simulink model "FAFA_Simulation"  (R2024b)
settings: Solver=FixedStepAuto  StartTime=0.0  StopTime=250  FixedStep=0.1  RelTol=1e-3
model workspace (MAT data in the model file):
  E = 0
  N = 0
  U = 70
  a_lat = [-2.8994  0.2017  -1.4522  -1.3994; -3.7694  1.1605  0.9879  -0.5752; 4.8979  -2.4536  -4.2099  -0.5761; 0.9075  1.8506  6.4665  2.8087]
  a_lon = [-0.1636  -0.7164  0.3908  0.5329; 0.8185  -0.2899  2.1971  2.5997; -0.1448  -2.0395  -0.2446  1.4062; 0.6823  -2.5415  -6.117  -5.7482]
  b_lat = [-2.6641  1.8404; -6.8743  1.3852; 17.3529  -0.0089; -11.8089  -3.3692]
  b_lon = [1.3105; 2.2437; -0.9608; -9.211]
  c_lat = [-0.6923  0.0805  -0.3221  -0.3931; -1.1619  0.5751  1.1098  0.0833; 0.5476  0.4203  0.2079  -0.0052; -0.4273  0.7792  0.2479  -0.0005]
  c_lon = [-5.1576  -28.9963  19.7487  -10.7497; -0.0952  -0.3715  -0.0997  -0.0942; 0.5331  -3.4973  -0.5832  0.4945; 3.6707  -0.1414  -0.2256  -0.1149]
  d_lat = [0  0; 0  0; 0  0; 0  0]
  d_lon = [0; 0; 0; 0]
  psi0 = 0
  wind_E0 = 0
  wind_N0 = 0
  wind_heading = 100
  wind_noise = 0
  wind_turbulance_value0 = 1
  wind_value0 = 0
  x0_lat = [0; 0; 0; 0]
  x0_lon = [0; 0; 0; 0]
undefined symbols (not defined in the file): dspblkCoreblockFVToolHelper, F, gcbh, Light, MIL, velocity, waypoints
libraries: simulink x8, slpidlib x5, aerolibwind2 x3, sharedtransform x2, rllib x1, uavutilslib x1
(part 1 of 3)
settings Model: PacingRate=3  Creator=user  LastModifiedBy=yeyi5
settings DataIOCC: SaveOutput=off  SignalLogging=off  DSMLogging=off  SaveTime=off
settings OptimizationCC: ReuseModelBlockBuffer=off
settings DebuggingCC: AlgebraicLoopMsg=none  ArtificialAlgebraicLoopMsg=none  InheritedTsInSrcMsg=none  TasksWithSamePriorityMsg=none  SigSpecEnsureSampleTimeMsg=none  UnconnectedLineMsg=warning  UnknownTsInhSupMsg=none  ModelReferenceDataLoggingMessage=none  OperatingPointInterfaceChecksumMismatchMsg=none  SFUnusedDataAndEventsDiag=none  SFTransitionActionBeforeConditionDiag=none  IntegerSaturationMsg=none
settings ModelReferenceCC: EnableRefExpFcnMdlSchedulingChecks=on
settings RTWCC: GPUComputeCapability=3.5  DLArmComputeVersion=19.05

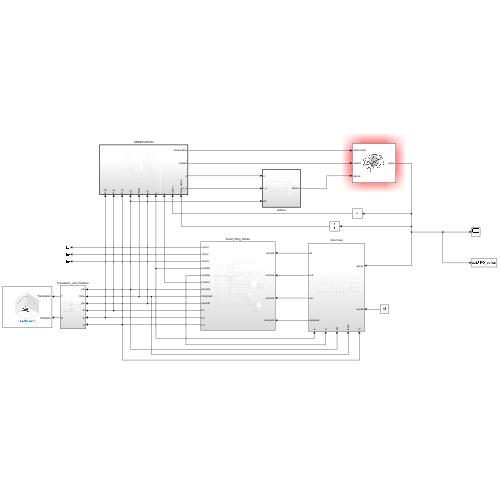
[thumbnail: Simulink's stored preview of the top-level diagram]
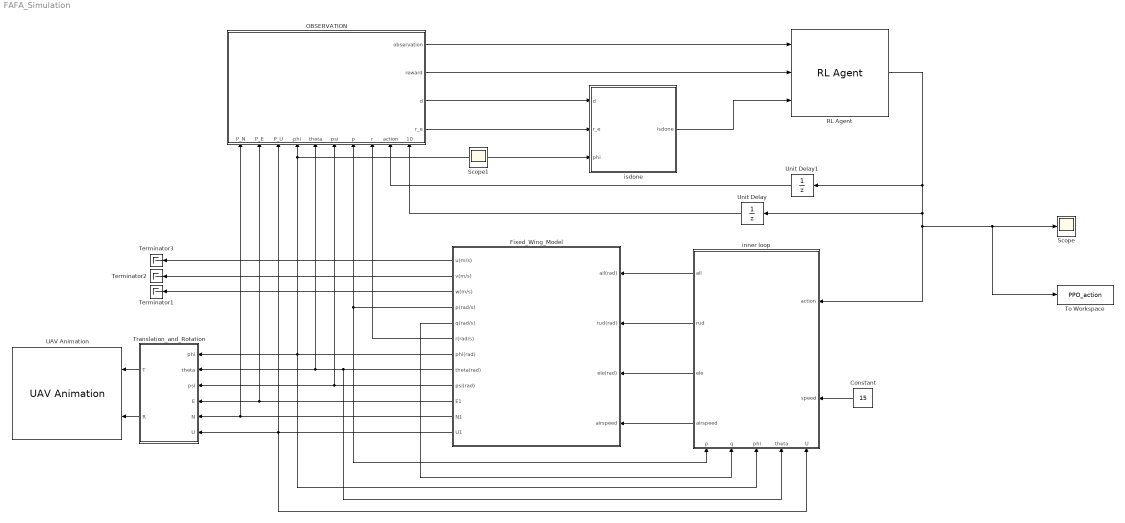
== system FAFA_Simulation ==
  Constant : Constant  Value=15
  Fixed_Wing_Model : Subsystem
  OBSERVATION : Subsystem  TreatAsAtomicUnit=on
      settings: PortSchema="{\"entries\":[{\"content\":{\"sides\":[{\"content\":{},\"type\":\"ConnectorPlacement.EquallySpacedRectSide\",\"uuid\":\"f286f6f9-a01a-42a6-836e-b598d67e253d\"},{\"content\":{\"connectorIds\":[\"Out1\",\"Out2\",\"Out3\",\"Out4\"],\"side\":\"RIGHT\"},\"type\":\"ConnectorPlacement.EquallySpacedRectSide\",\"uuid\":\"2d728f1a-8a2e-4ecd-bbb7-96377896084d\"},{\"content\":{\"side\":\"TOP\"},\"type\":\"ConnectorPlacement.EquallySpacedRectSide\",\"uuid\":\"cacb8353-56c3-4403-9fcf-3680ca0986aa\"},{\"content\":{\"connectorIds\":[\"In1\",\"In2\",\"In3\",\"In4\",\"In5\",\"In6\",\"In7\",\"In8\",\"In9\",\"In10\"],\"side\":\"BOTTOM\"},\"type\":\"ConnectorPlacement.EquallySpacedRectSide\",\"uuid\":\"73d02477-6798-4d99-8273-17e2202a1dc5\"}]},\"type\":\"ConnectorPlacement.EquallySpacedConnector\",\"uuid\":\"e5ed1a66-3715-4ac1-9ed0-cc3d392d34e5\"}],\"packageUris\":[\"http://schema.mathworks.com/mf0/Connector/R2020b\"],\"version\":\"1.0\"}"
  RL Agent : rllib/RL Agent  Agent=Agent_Stage2  ExternalActionAsInput=off  ProvideLastAction=off  ProvideCumRwd=off  TreatAsDirectFeedthrough=on  UseStrictObservationDataTypes=off
  Scope : Scope
  Terminator1 : Terminator
  Terminator2 : Terminator
  Terminator3 : Terminator
  To Workspace : ToWorkspace  VariableName=PPO_action  SaveFormat=Timeseries  SampleTime=-1
  Translation_and_Rotation : Subsystem
  UAV Animation : uavutilslib/UAV Animation  NumUAV=1  DynamicUAVConfig=off  UAVType=FixedWing  UAVSize=50  UAVColor=[1 0 0]  UAVTrajectoryAlpha=1  InertialZDirection=Up  RotationFormat=Quaternion  DrawMarkers=off  SampleTime=0.1
  Unit Delay : UnitDelay  SampleTime=0.2  HasFrameUpgradeWarning=on
  Unit Delay1 : UnitDelay  SampleTime=0.1  HasFrameUpgradeWarning=on
  inner loop : Subsystem
      settings: PortSchema="{\"entries\":[{\"content\":{\"sides\":[{\"content\":{\"connectorIds\":[\"In1\",\"In2\"]},\"type\":\"ConnectorPlacement.EquallySpacedRectSide\",\"uuid\":\"7d60b91c-7846-4215-9a9d-48d8590b6647\"},{\"content\":{\"connectorIds\":[\"Out1\",\"Out2\",\"Out3\",\"Out4\"],\"side\":\"RIGHT\"},\"type\":\"ConnectorPlacement.EquallySpacedRectSide\",\"uuid\":\"9adb366d-c473-491f-8767-4ec8db5c324b\"},{\"content\":{\"connectorIds\":[\"In3\",\"In4\",\"In5\",\"In6\",\"In7\"],\"side\":\"TOP\"},\"type\":\"ConnectorPlacement.EquallySpacedRectSide\",\"uuid\":\"05cfcaa8-de81-40d5-bf1e-81a0cec58454\"},{\"content\":{\"side\":\"BOTTOM\"},\"type\":\"ConnectorPlacement.EquallySpacedRectSide\",\"uuid\":\"953cf2cb-5cfd-4159-a7f8-9598cb97629a\"}]},\"type\":\"ConnectorPlacement.EquallySpacedConnector\",\"uuid\":\"4935b2dc-fa79-4ba1-b3ea-575a125b9ddc\"}],\"packageUris\":[\"http://schema.mathworks.com/mf0/Connector/R2020b\"],\"version\":\"1.0\"}"
  isdone : Subsystem  TreatAsAtomicUnit=on
  Scope1 : Scope
  wires:
  Translation_and_Rotation/2(R) -> UAV Animation/2
  Translation_and_Rotation/1(T) -> UAV Animation/1
  Fixed_Wing_Model/3(w(m/s)) -> Terminator1/1
  Fixed_Wing_Model/2(v(m/s)) -> Terminator2/1
  Fixed_Wing_Model/1(u(m/s)) -> Terminator3/1
  RL Agent/1 -> Unit Delay1/1, Scope/1, To Workspace/1, inner loop/2(action), Unit Delay/1
  OBSERVATION/2(reward) -> RL Agent/2
  OBSERVATION/1(observation) -> RL Agent/1
  OBSERVATION/3(d) -> isdone/1(d)
  OBSERVATION/4(r_e) -> isdone/2(r_e)
  Fixed_Wing_Model/4(p(rad/s)) -> inner loop/7(p), OBSERVATION/7(p)
  Fixed_Wing_Model/5(q(rad/s)) -> inner loop/6(q)
  Fixed_Wing_Model/6(r(rad/s)) -> OBSERVATION/8(r)
  Fixed_Wing_Model/7(phi(rad)) -> inner loop/5(phi), Translation_and_Rotation/1(phi), isdone/3(phi), OBSERVATION/4(phi)
  Fixed_Wing_Model/8(theta(rad)) -> OBSERVATION/5(theta), Translation_and_Rotation/2(theta), inner loop/4(theta)
  Fixed_Wing_Model/9(psi(rad)) -> Translation_and_Rotation/3(psi), OBSERVATION/6(psi)
  Fixed_Wing_Model/10(E1) -> Translation_and_Rotation/4(E), OBSERVATION/2(P_E)
  Fixed_Wing_Model/11(N1) -> Translation_and_Rotation/5(N), OBSERVATION/1(P_N)
  Fixed_Wing_Model/12(U1) -> inner loop/3(U), Translation_and_Rotation/6(U), OBSERVATION/3(P_U)
  Unit Delay1/1 -> OBSERVATION/9(action)
  Unit Delay/1 -> OBSERVATION/10(delay_action)
  inner loop/4(ail) -> Fixed_Wing_Model/1(ail(rad))
  inner loop/3(rud) -> Fixed_Wing_Model/2(rud(rad))
  inner loop/2(ele) -> Fixed_Wing_Model/3(ele(rad))
  inner loop/1(airspeed) -> Fixed_Wing_Model/4(airspeed)
  Constant/1 -> inner loop/1(speed)
  isdone/1(isdone) -> RL Agent/3

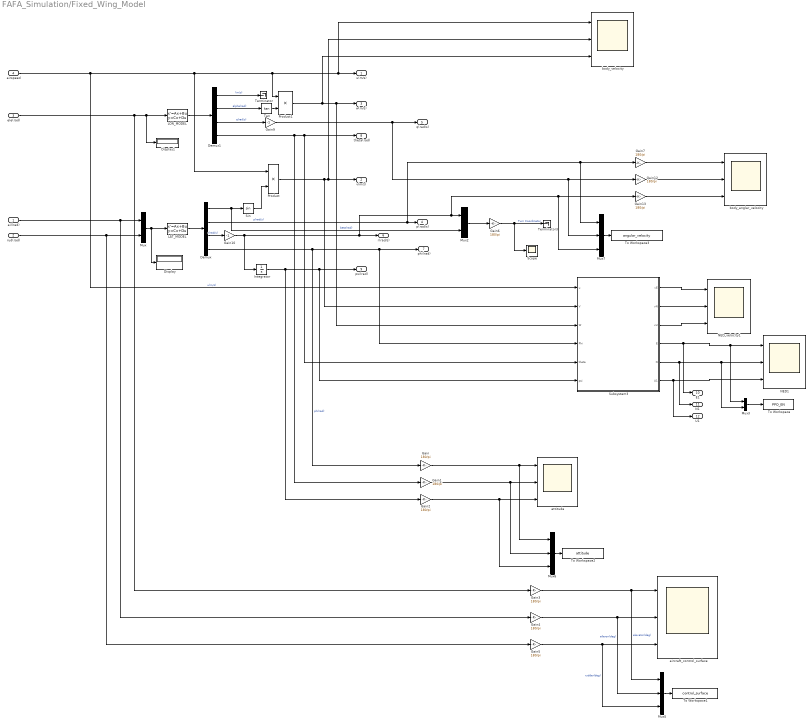
== system FAFA_Simulation/Fixed_Wing_Model ==
  ail(rad) : Inport
  rud(rad) : Inport  Port=2
  ele(rad) : Inport  Port=3
  airspeed : Inport  Port=4
  Demux : Demux
  Demux1 : Demux
  Display : Display
  Display1 : Display
  Gain{,1..7,12..13} (10 alike) : Gain  Gain=180/pi
  Gain10 : Gain  Gain=-1
  Gain9 : Gain  Gain=-1
  Integrator : Integrator  InitialCondition=psi0  WrapState=on
  LAT_MODEL : StateSpace  A=a_lat  B=b_lat  C=c_lat  D=d_lat  InitialCondition=x0_lat
  LON_MODEL : StateSpace  A=a_lon  B=b_lon  C=c_lon  D=d_lon  InitialCondition=x0_lon
  Mux : Mux  Inputs=2
  Mux2 : Mux  Inputs=2
  Mux3 : Mux  Inputs=2
  Mux5 : Mux  Inputs=3
  Mux6 : Mux  Inputs=3
  Mux7 : Mux  Inputs=3
  NED1 : Scope  NumInputPorts=3
  NED_velocity1 : Scope  NumInputPorts=3
  Product : Product
  Product1 : Product
  Scope : Scope
  Sin : Trigonometry
  Subsystem3 : Subsystem
  Tan : Trigonometry  Operator=tan
  Terminator : Terminator
  Terminator3 : Terminator
  To Workspace : ToWorkspace  VariableName=PPO_EN  SaveFormat=Timeseries  SampleTime=-1
  To Workspace1 : ToWorkspace  VariableName=control_surface  SaveFormat=Timeseries  SampleTime=-1
  To Workspace2 : ToWorkspace  VariableName=attitude  SaveFormat=Timeseries  SampleTime=-1
  To Workspace3 : ToWorkspace  VariableName=angular_velocity  SaveFormat=Timeseries  SampleTime=-1
  aircraft_control_surface : Scope  NumInputPorts=3
  attitude : Scope  NumInputPorts=3
  body_anglar_velocity : Scope  NumInputPorts=3
  body_velocity : Scope  NumInputPorts=3
  u(m/s) : Outport
  v(m/s) : Outport  Port=2
  w(m/s) : Outport  Port=3
  p(rad/s) : Outport  Port=4
  q(rad/s) : Outport  Port=5
  r(rad/s) : Outport  Port=6
  phi(rad) : Outport  Port=7
  theta(rad) : Outport  Port=8
  psi(rad) : Outport  Port=9
  E1 : Outport  Port=10
  N1 : Outport  Port=11
  U1 : Outport  Port=12
  wires:
  Demux/3 -> Gain10/1  "r(rad/s)"
  Mux/1 -> Display/1, LAT_MODEL/1
  LON_MODEL/1 -> Demux1/1
  Demux/1 -> Sin/1, Mux2/2  "beta(rad)"
  LAT_MODEL/1 -> Demux/1
  Demux/2 -> Mux7/1, Gain7/1, p(rad/s)/1  "p(rad/s)"
  airspeed/1 -> Subsystem3/1(u), body_velocity/1, u(m/s)/1, Product1/1, Product/1  "u(m/s)"
  Sin/1 -> Product/2
  Demux1/1 -> Terminator/1  "(m/s)"
  Demux1/2 -> Tan/1  "alpha(rad)"
  Demux1/3 -> Gain9/1  "q(rad/s)"
  Tan/1 -> Product1/2
  Gain/1 -> Mux6/1, attitude/1
  Gain1/1 -> Mux6/2, attitude/2
  Gain5/1 -> Mux5/3, aircraft_control_surface/3  "rudder(deg)"
  Gain3/1 -> Mux5/1, aircraft_control_surface/1  "elevator(deg)"
  Gain4/1 -> Mux5/2, aircraft_control_surface/2  "aileron(deg)"
  Mux5/1 -> To Workspace1/1
  Mux6/1 -> To Workspace2/1
  Mux7/1 -> To Workspace3/1
  Mux2/1 -> Gain6/1
  Gain6/1 -> Scope/1, Terminator3/1  "Turn Coordinator"
  Demux/4 -> Subsystem3/4(Phi), phi(rad)/1, Gain/1  "phi(rad)"
  Subsystem3/1(vE) -> NED_velocity1/1
  Subsystem3/2(vN) -> NED_velocity1/2
  Subsystem3/3(vU) -> NED_velocity1/3
  Gain9/1 -> Mux7/2, Gain12/1, q(rad/s)/1
  Gain2/1 -> Mux6/3, attitude/3
  Mux3/1 -> To Workspace/1
  Integrator/1 -> Subsystem3/6(psi), psi(rad)/1, Gain2/1
  Gain10/1 -> r(rad/s)/1, Mux7/3, Gain13/1, Mux2/1, Integrator/1
  Gain7/1 -> body_anglar_velocity/1
  Gain12/1 -> body_anglar_velocity/2
  Gain13/1 -> body_anglar_velocity/3
  ail(rad)/1 -> Gain4/1, Mux/1
  rud(rad)/1 -> Gain5/1, Mux/2
  Subsystem3/4(E) -> E1/1, Mux3/1, NED1/1
  Subsystem3/5(N) -> N1/1, Mux3/2, NED1/2
  Subsystem3/6(U1) -> U1/1, NED1/3
  Product/1 -> Subsystem3/2(V), v(m/s)/1, body_velocity/2
  Product1/1 -> body_velocity/3, Subsystem3/3(W), w(m/s)/1
  Demux1/4 -> theta(rad)/1, Subsystem3/5(theta), Gain1/1
  ele(rad)/1 -> Gain3/1, Display1/1, LON_MODEL/1

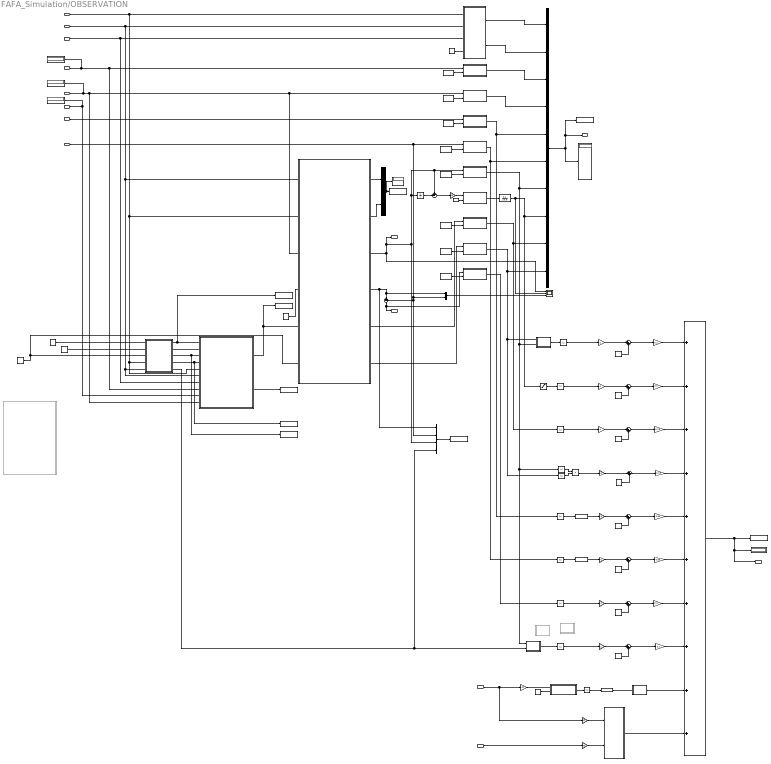
== system FAFA_Simulation/OBSERVATION ==
  P_N : Inport
  P_E : Inport  Port=2
  P_U : Inport  Port=3
  phi : Inport  Port=4
  theta : Inport  Port=5
  psi : Inport  Port=6
  p : Inport  Port=7
  r : Inport  Port=8
  action : Inport  Port=9
  delay_action : Inport  Port=10
  Abs{1,3..5,10..13,15,17} (10 alike) : Abs  SaturateOnIntegerOverflow=off
  Compare To Constant2 : simulink/Logic and Bit Operations/Compare To Constant  relop=>=  const=0.5  OutDataTypeStr=boolean
  Compare To Constant5 : simulink/Logic and Bit Operations/Compare To Constant  relop=>=  const=0.5  OutDataTypeStr=boolean
  Compare To Constant7 : simulink/Logic and Bit Operations/Compare To Constant  relop=>  const=1  OutDataTypeStr=boolean
  Constant : Constant  Value=15
  Constant1 : Constant  Value=60*pi/180
  Constant10 : Constant  Value=30
  Constant11 : Constant  Value=6
  Constant12 : Constant  Value=pi
  Constant{13,16,18..22,24} (8 alike) : Constant
  Constant14 : Constant  Value=1/55
  Constant15 : Constant  Value=25*pi/180
  Constant2 : Constant  Value=60*pi/180
  Constant27 : Constant  Value=40
  Constant4 : Constant  Value=100
  Constant7 : Constant  Value=0.01
  Constant8 : Constant  Value=40*pi/180
  Constant9 : Constant  Value=pi/2
  Discrete Transfer Fcn : DiscreteTransferFcn  LoadFcn=dspblkCoreblockFVToolHelper(gcbh,'load');  Numerator=[0.2]  Denominator=[1, -0.8]
      settings: CopyFcn=dspblkCoreblockFVToolHelper(gcbh,'copy');  DeleteFcn=dspblkCoreblockFVToolHelper(gcbh,'close');  ModelCloseFcn=dspblkCoreblockFVToolHelper(gcbh,'close');  PreSaveFcn=dspblkCoreblockFVToolHelper(gcbh,'presave');  PostSaveFcn=dspblkCoreblockFVToolHelper(gcbh,'postsave');  CloseFcn=dspblkCoreblockFVToolHelper(gcbh,'close');
  Display{,1..5} (6 alike) : Display
  Gain{1,10,14..16,21..22} (7 alike) : Gain  Gain=-1
  Gain11 : Gain  Gain=0.1
  Gain12 : Gain
  Gain13 : Gain  Gain=0.1
  Gain17 : Gain  Gain=0.15
  Gain18 : Gain  Gain=0.05
  Gain19 : Gain  Gain=0.2
  Gain20 : Gain  Gain=0.15
  Gain23 : Gain  Gain=0.05
  Gain4 : Gain  Gain=40
  Gain5 : Gain  Gain=40
  Gain6 : Gain  Gain=40
  Gain8 : Gain  Gain=10
  Gain9 : Gain  Gain=0.2
  MATLAB Function1 : MATLAB Function  TreatAsAtomicUnit=on
  MATLAB Function10 : MATLAB Function  TreatAsAtomicUnit=on
  MATLAB Function11 : MATLAB Function  TreatAsAtomicUnit=on
  MATLAB Function12 : MATLAB Function  TreatAsAtomicUnit=on  SystemSampleTime=0.1
  MATLAB Function13 : MATLAB Function  TreatAsAtomicUnit=on
  MATLAB Function14 : MATLAB Function  Commented=on  TreatAsAtomicUnit=on
  MATLAB Function15 : MATLAB Function  TreatAsAtomicUnit=on
  MATLAB Function16 : MATLAB Function  TreatAsAtomicUnit=on
  MATLAB Function18 : MATLAB Function  TreatAsAtomicUnit=on
  MATLAB Function2 : MATLAB Function  TreatAsAtomicUnit=on
  MATLAB Function20 : MATLAB Function  TreatAsAtomicUnit=on
  MATLAB Function21 : MATLAB Function  Commented=on  TreatAsAtomicUnit=on
  MATLAB Function22 : MATLAB Function  TreatAsAtomicUnit=on
  MATLAB Function3 : MATLAB Function  TreatAsAtomicUnit=on  SystemSampleTime=0.1
  MATLAB Function4 : MATLAB Function  TreatAsAtomicUnit=on
  MATLAB Function5 : MATLAB Function  TreatAsAtomicUnit=on
  MATLAB Function6 : MATLAB Function  TreatAsAtomicUnit=on
  MATLAB Function7 : MATLAB Function  TreatAsAtomicUnit=on
  MATLAB Function8 : MATLAB Function  TreatAsAtomicUnit=on  SystemSampleTime=0.1
  MATLAB Function9 : MATLAB Function  TreatAsAtomicUnit=on
  Mux : Mux  Inputs=10
  Mux1 : Mux  Inputs=2
  Mux2 : Mux
  Mux3 : Mux  Inputs=2
  Product : Product
  Saturation : Saturate  UpperLimit=1  LowerLimit=-1
  Straight Line V4 : MATLAB Function  Commented=on  TreatAsAtomicUnit=on  SystemSampleTime=0.1
  Sum : Sum  Inputs=|+-
  Sum{4..5,7,10..14} (8 alike) : Sum  Inputs=|++
  Sum3 : Sum  Inputs=++++++++++
  Sum6 : Sum  Inputs=+-|
  To Workspace1 : ToWorkspace  VariableName=PPO_ref_EN  SaveFormat=Timeseries  SampleTime=-1
  To Workspace2 : ToWorkspace  VariableName=SPSO_path  SaveFormat=Timeseries  SampleTime=-1
  To Workspace3 : ToWorkspace  VariableName=Reward  SaveFormat=Timeseries  SampleTime=-1
  To Workspace4 : ToWorkspace  VariableName=observation  SaveFormat=Timeseries  SampleTime=-1
  To Workspace5 : ToWorkspace  VariableName=valid_flag  SaveFormat=Timeseries  SampleTime=-1
  To Workspace6 : ToWorkspace  VariableName=loiter_flag  SaveFormat=Timeseries  SampleTime=-1
  To Workspace7 : ToWorkspace  VariableName=target_trajectory  SaveFormat=Timeseries  SampleTime=-1
  To Workspace8 : ToWorkspace  VariableName=guidance_error  SaveFormat=Timeseries  SampleTime=-1
  To Workspace9 : ToWorkspace  VariableName=guidance_mode  SaveFormat=Timeseries  SampleTime=-1
  Unit Delay : UnitDelay  SampleTime=0.1  HasFrameUpgradeWarning=on
  guidance_error : Scope  NumInputPorts=3
  velocity : Constant  Value=velocity
  waypoints : Constant  Value=waypoints
  observation : Outport
  reward : Outport  Port=2
  d : Outport  Port=3
  r_e : Outport  Port=4
  wires:
  Gain15/1 -> Sum10/1
  Sum10/1 -> Gain9/1
  Abs10/1 -> Gain15/1  "d"
  Constant18/1 -> Sum10/2
  Gain16/1 -> Sum11/1
  Sum11/1 -> Gain17/1
  Constant20/1 -> Sum11/2
  Abs11/1 -> Gain16/1  "heta"
  Gain22/1 -> Sum14/1
  Constant24/1 -> Sum14/2
  Sum14/1 -> Gain23/1
  Compare To Constant7/1 -> MATLAB Function20/1(bool)
  Constant27/1 -> MATLAB Function18/2(Finite)
  action/1 -> Gain4/1, Gain5/1
  Abs17/1 -> Compare To Constant7/1
  MATLAB Function18/1(y) -> Abs17/1
  Sum3/1 -> reward/1, Display2/1, To Workspace3/1
  Gain4/1 -> MATLAB Function18/1(x)
  Gain5/1 -> MATLAB Function16/1(roll)
  Constant/1 -> MATLAB Function12/4(v)
  psi/1 -> MATLAB Function12/3(psi), MATLAB Function7/1(x), MATLAB Function8/10(uav_psi), Display4/1
  Constant10/1 -> MATLAB Function1/2(finite)
  MATLAB Function12/3(d) -> guidance_error/1, d/1, Sum6/1, MATLAB Function1/1(x), Unit Delay/1, Mux2/3  "d"
  Constant2/1 -> MATLAB Function4/2(finite)
  MATLAB Function4/1(y) -> Abs5/1, Mux/6  "r"
  r/1 -> MATLAB Function4/1(x), Mux1/2, Mux2/2, Sum/2
  Constant1/1 -> MATLAB Function2/2(finite)
  MATLAB Function2/1(y) -> Abs15/1, Mux/5  "p"
  p/1 -> MATLAB Function2/1(x)
  Constant8/1 -> MATLAB Function6/2(finite)
  MATLAB Function6/1(y) -> Mux/3  "phi"
  phi/1 -> MATLAB Function8/8(uav_phi), MATLAB Function6/1(x), Display/1
  Constant9/1 -> MATLAB Function7/2(finite)
  MATLAB Function7/1(y) -> Mux/4  "psi"
  Constant12/1 -> MATLAB Function9/2(finite)
  MATLAB Function9/1(y) -> Mux/9, Abs11/1  "heta"
  Constant14/1 -> MATLAB Function11/2(finite)
  MATLAB Function12/5(heta) -> MATLAB Function9/1(x)  "heta"
  MATLAB Function12/6(curvature) -> MATLAB Function11/1(x)  "curvaure"
  Sum4/1 -> Gain11/1
  Abs3/1 -> Gain12/1
  Gain12/1 -> Sum4/1
  Constant19/1 -> Sum4/2
  MATLAB Function22/1(y) -> Abs3/1
  MATLAB Function16/1(r_roll) -> Sum3/10
  MATLAB Function20/1(y) -> Sum3/9
  Gain11/1 -> Sum3/8
  Gain23/1 -> Sum3/5
  Gain20/1 -> Sum3/4
  Gain17/1 -> Sum3/3
  Gain9/1 -> Sum3/1
  Mux3/1 -> Display1/1, To Workspace1/1
  Mux/1 -> To Workspace4/1, observation/1, Display3/1
  MATLAB Function12/4(delta_psi) -> Mux2/1, Sum/1, Mux1/1  "ref_r"
  Sum/1 -> MATLAB Function15/1(x), r_e/1
  P_U/1 -> MATLAB Function8/7(uav_u), MATLAB Function5/3(P_U)
  Mux1/1 -> guidance_error/3
  Gain6/1 -> MATLAB Function16/2(roll_d)
  delay_action/1 -> Gain6/1
  Sum6/1 -> Gain8/1
  Constant11/1 -> MATLAB Function10/2(finite)
  MATLAB Function10/1(y) -> Discrete Transfer Fcn/1  "d_dot"
  Unit Delay/1 -> Sum6/2
  Gain8/1 -> MATLAB Function10/1(x)  "d_dot"
  Constant13/1 -> Sum5/2
  Abs4/1 -> Gain10/1  "d_dot"
  Saturation/1 -> Abs4/1
  Gain10/1 -> Sum5/1
  Sum5/1 -> Gain13/1
  Gain13/1 -> Sum3/2
  Abs15/1 -> Compare To Constant5/1  "p"
  Compare To Constant5/1 -> Gain22/1
  Abs5/1 -> Compare To Constant2/1  "r"
  Gain14/1 -> Sum7/1
  Constant16/1 -> Sum7/2
  Sum7/1 -> Gain18/1
  Gain18/1 -> Sum3/6
  Compare To Constant2/1 -> Gain14/1
  Discrete Transfer Fcn/1 -> guidance_error/2, Saturation/1, Mux/8  "d_dot"
  MATLAB Function3/3(valid_flag) -> To Workspace5/1, MATLAB Function8/3(valid_flag)
  MATLAB Function3/4(loiter_flag) -> To Workspace6/1, MATLAB Function8/4(loiter_flag)
  MATLAB Function12/1(E) -> Mux3/1
  MATLAB Function12/2(N) -> Mux3/2  "N"
  MATLAB Function13/1(y) -> Abs10/1
  P_E/1 -> MATLAB Function5/1(P_E), MATLAB Function8/5(uav_e), MATLAB Function3/4(uav_e), MATLAB Function12/2(P_E)
  P_N/1 -> MATLAB Function8/6(uav_n), MATLAB Function3/5(uav_n), MATLAB Function12/1(P_N), MATLAB Function5/2(P_N)
  Constant7/1 -> MATLAB Function5/4(alpha)
  MATLAB Function5/1(P_E_norm) -> Mux/1
  MATLAB Function5/2(P_N_norm) -> Mux/2
  MATLAB Function3/5(distance_to_target) -> MATLAB Function22/2(dis), Mux2/4
  Mux2/1 -> To Workspace8/1
  MATLAB Function15/1(y) -> Abs12/1  "r_e"
  Constant15/1 -> MATLAB Function15/2(finite)
  Gain1/1 -> Sum12/1
  Abs12/1 -> Gain1/1  "r_e"
  Constant21/1 -> Sum12/2
  Sum12/1 -> Gain19/1
  Gain19/1 -> Sum3/7
  Gain21/1 -> Sum13/1
  Abs1/1 -> Product/2  "kt"
  Product/1 -> Gain21/1
  MATLAB Function1/1(y) -> MATLAB Function22/1(d), Abs13/1, MATLAB Function13/2(d), Mux/7  "d"
  Sum13/1 -> Gain20/1
  MATLAB Function11/1(y) -> Mux/10, Abs1/1, MATLAB Function13/1(kt)  "kt"
  Abs13/1 -> Product/1  "d"
  Constant22/1 -> Sum13/2
  MATLAB Function3/2(velocity_window) -> MATLAB Function8/2(velocity_window)
  MATLAB Function3/1(waypoints_window) -> To Workspace7/1, MATLAB Function8/1(waypoints_window)
  velocity/1 -> MATLAB Function3/2(velocity_in)
  waypoints/1 -> MATLAB Function3/1(position_in)
  MATLAB Function8/2(guidance_mode) -> To Workspace9/1
  theta/1 -> MATLAB Function8/9(uav_theta), Display5/1
  MATLAB Function8/1(global_path) -> To Workspace2/1, MATLAB Function12/5(path)
  Constant4/1 -> MATLAB Function12/6(windowLen), MATLAB Function3/3(window_length)

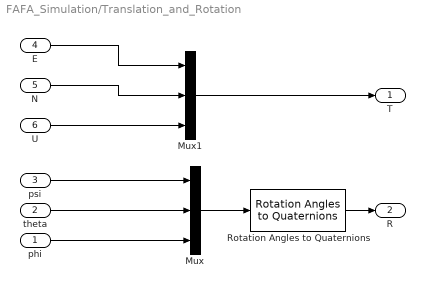
== system FAFA_Simulation/Translation_and_Rotation ==
  phi : Inport
  theta : Inport  Port=2
  psi : Inport  Port=3
  E : Inport  Port=4
  N : Inport  Port=5
  U : Inport  Port=6
  Mux : Mux  Inputs=3
  Mux1 : Mux  Inputs=3
  Rotation Angles to Quaternions : sharedtransform/Rotation Angles to Quaternions  rotationOrder=ZYX  aMode=aMode
  T : Outport
  R : Outport  Port=2
  wires:
  Mux/1 -> Rotation Angles to Quaternions/1
  Rotation Angles to Quaternions/1 -> R/1
  Mux1/1 -> T/1
  U/1 -> Mux1/3
  psi/1 -> Mux/1
  theta/1 -> Mux/2
  phi/1 -> Mux/3
  E/1 -> Mux1/1
  N/1 -> Mux1/2

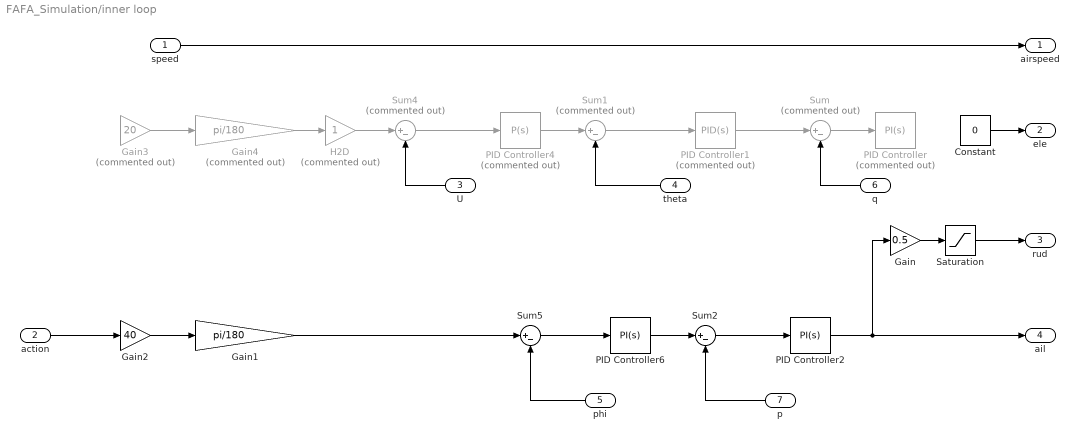
== system FAFA_Simulation/inner loop ==
  speed : Inport
  action : Inport  Port=2
  U : Inport  Port=3
  theta : Inport  Port=4
  phi : Inport  Port=5
  q : Inport  Port=6
  p : Inport  Port=7
  Constant : Constant  Value=0
  Gain : Gain  Gain=0.5
  Gain1 : Gain  Gain=pi/180
  Gain2 : Gain  Gain=40
  Gain3 : Gain  Commented=on  Gain=20
  Gain4 : Gain  Commented=on  Gain=pi/180
  H2D : Gain  Commented=on
  PID Controller : slpidlib/PID Controller  Commented=on  Controller=PI  Form=Parallel  TimeDomain=Continuous-time  UseExternalTs=off  SampleTime=-1  IntegratorMethod=Forward Euler  FilterMethod=Forward Euler  ControllerParametersSource=internal  P=0.0379742774014741  I=0.434388894979822  UseKiTs=off  D=0  UseExternalDerivativeSource=off  N=100  UseFilter=on  TunerSelectOption=Transfer Function Based (PID Tuner App)  InitialConditionSource=internal  InitialConditionForIntegrator=0  InitialConditionForFilter=0  DifferentiatorICPrevScaledInput=0  ExternalReset=none  TrackingMode=off  Kt=1  LimitOutput=on  SatLimitsSource=internal  UpperSaturationLimit=12*(pi/180)  LowerSaturationLimit=-12*(pi/180)  LinearizeAsGain=on  AntiWindupMode=none  Kb=1  LimitIntegrator=off  UpperIntegratorSaturationLimit=inf  LowerIntegratorSaturationLimit=-inf  POutMin=[]  POutMax=[]  IOutMin=[]  IOutMax=[]  DOutMin=[]  DOutMax=[]  NOutMin=[]  NOutMax=[]  SumOutMin=[]  SumOutMax=[]  SaturationOutMin=[]  SaturationOutMax=[]  PParamMin=[]  PParamMax=[]  IParamMin=[]  IParamMax=[]  DParamMin=[]  DParamMax=[]  NParamMin=[]  NParamMax=[]  KbParamMin=[]  KbParamMax=[]  KtParamMin=[]  KtParamMax=[]  KbOutMin=[]  KbOutMax=[]  KtOutMin=[]  KtOutMax=[]  IntegratorOutMin=[]  IntegratorOutMax=[]  FilterOutMin=[]  FilterOutMax=[]  SumI1OutMin=[]  SumI1OutMax=[]  SumI2OutMin=[]  SumI2OutMax=[]  SumI3OutMin=[]  SumI3OutMax=[]  SumI4OutMin=[]  SumI4OutMax=[]  SumDOutMin=[]  SumDOutMax=[]  DifferentiatorOutMin=[]  DifferentiatorOutMax=[]  FilterDiffOutCoefMin=[]  FilterDiffOutCoefMax=[]  ReciprocalOutMin=[]  ReciprocalOutMax=[]  SumDenOutMin=[]  SumDenOutMax=[]  SumNumOutMin=[]  SumNumOutMax=[]  DivideOutMin=[]  DivideOutMax=[]  UdiffTsProdOutMin=[]  UdiffTsProdOutMax=[]  NTsProdOutMin=[]  NTsProdOutMax=[]  UintegralTsProdOutMin=[]  UintegralTsProdOutMax=[]  UngainTsProdOutMin=[]  UngainTsProdOutMax=[]  ClampingZeroOutDataTypeStr=Inherit: Inherit via back propagation  ClampingZeroOutMin=[]  ClampingZeroOutMax=[]  FilterDenConstantOutDataTypeStr=Inherit: Inherit via back propagation  FilterDenConstantOutMin=[]  FilterDenConstantOutMax=[]  PCopyOutDataTypeStr=Inherit: Inherit via back propagation  PCopyOutMin=[]  PCopyOutMax=[]  NCopyOutDataTypeStr=Inherit: Inherit via back propagation  NCopyOutMin=[]  NCopyOutMax=[]  IntegratorContinuousStateAttributes=''  IntegratorStateMustResolveToSignalObject=off  IntegratorRTWStateStorageClass=Auto  FilterContinuousStateAttributes=''  FilterStateMustResolveToSignalObject=off  FilterRTWStateStorageClass=Auto  ParallelPVariant=InternalParameters  IdealPVariant=Disabled  IVariant=InternalParameters  DVariant=Disabled  IntegratorVariant=Continuous  SatVariant=Enabled  AWVariant=Passthrough  PCopyVariant=Disabled  TRVariant=Disabled  FdbkBlocksVariant=Forward  IdealPFdbkVariant=Disabled  SatFdbkVariant=Disabled  DerivativeFilterVariant=Disabled  NVariant=Disabled  NCopyVariant=Disabled_SignalSpec  FilterICVariant=Disabled  IntegratorICVariant=InternalICs  ExternalResetVariant=Disabled  TRSumVariant=Passthrough  SumFdbkVariant=Disabled  SumVariant=Sum_PI  TsampFilterVariant=InternalTs  TsampNgainVariant=Passthrough  TsampIntegralVariant=Disabled_SignalSpec  ExternalSaturationOutDataTypeStr=Inherit: Same as second input  DerivativeSourceVariant=Disabled  PreIntVariant=InternalPreInt
  PID Controller1 : slpidlib/PID Controller  Commented=on  Controller=PID  Form=Parallel  TimeDomain=Continuous-time  UseExternalTs=off  SampleTime=-1  IntegratorMethod=Forward Euler  FilterMethod=Forward Euler  ControllerParametersSource=internal  P=0.172177541949498  I=0.00749662716740607  UseKiTs=off  D=-0.106148159358307  UseExternalDerivativeSource=off  N=1.62204924692388  UseFilter=on  TunerSelectOption=Transfer Function Based (PID Tuner App)  InitialConditionSource=internal  InitialConditionForIntegrator=0  InitialConditionForFilter=0  DifferentiatorICPrevScaledInput=0  ExternalReset=none  TrackingMode=off  Kt=1  LimitOutput=on  SatLimitsSource=internal  UpperSaturationLimit=60*(pi/180)  LowerSaturationLimit=-60*(pi/180)  LinearizeAsGain=on  AntiWindupMode=none  Kb=1  LimitIntegrator=off  UpperIntegratorSaturationLimit=inf  LowerIntegratorSaturationLimit=-inf  POutMin=[]  POutMax=[]  IOutMin=[]  IOutMax=[]  DOutMin=[]  DOutMax=[]  NOutMin=[]  NOutMax=[]  SumOutMin=[]  SumOutMax=[]  SaturationOutMin=[]  SaturationOutMax=[]  PParamMin=[]  PParamMax=[]  IParamMin=[]  IParamMax=[]  DParamMin=[]  DParamMax=[]  NParamMin=[]  NParamMax=[]  KbParamMin=[]  KbParamMax=[]  KtParamMin=[]  KtParamMax=[]  KbOutMin=[]  KbOutMax=[]  KtOutMin=[]  KtOutMax=[]  IntegratorOutMin=[]  IntegratorOutMax=[]  FilterOutMin=[]  FilterOutMax=[]  SumI1OutMin=[]  SumI1OutMax=[]  SumI2OutMin=[]  SumI2OutMax=[]  SumI3OutMin=[]  SumI3OutMax=[]  SumI4OutMin=[]  SumI4OutMax=[]  SumDOutMin=[]  SumDOutMax=[]  DifferentiatorOutMin=[]  DifferentiatorOutMax=[]  FilterDiffOutCoefMin=[]  FilterDiffOutCoefMax=[]  ReciprocalOutMin=[]  ReciprocalOutMax=[]  SumDenOutMin=[]  SumDenOutMax=[]  SumNumOutMin=[]  SumNumOutMax=[]  DivideOutMin=[]  DivideOutMax=[]  UdiffTsProdOutMin=[]  UdiffTsProdOutMax=[]  NTsProdOutMin=[]  NTsProdOutMax=[]  UintegralTsProdOutMin=[]  UintegralTsProdOutMax=[]  UngainTsProdOutMin=[]  UngainTsProdOutMax=[]  ClampingZeroOutDataTypeStr=Inherit: Inherit via back propagation  ClampingZeroOutMin=[]  ClampingZeroOutMax=[]  FilterDenConstantOutDataTypeStr=Inherit: Inherit via back propagation  FilterDenConstantOutMin=[]  FilterDenConstantOutMax=[]  PCopyOutDataTypeStr=Inherit: Inherit via back propagation  PCopyOutMin=[]  PCopyOutMax=[]  NCopyOutDataTypeStr=Inherit: Inherit via back propagation  NCopyOutMin=[]  NCopyOutMax=[]  IntegratorContinuousStateAttributes=''  IntegratorStateMustResolveToSignalObject=off  IntegratorRTWStateStorageClass=Auto  FilterContinuousStateAttributes=''  FilterStateMustResolveToSignalObject=off  FilterRTWStateStorageClass=Auto  ParallelPVariant=InternalParameters  IdealPVariant=Disabled  IVariant=InternalParameters  DVariant=InternalParameters  IntegratorVariant=Continuous  SatVariant=Enabled  AWVariant=Passthrough  PCopyVariant=Disabled  TRVariant=Disabled  FdbkBlocksVariant=Forward  IdealPFdbkVariant=Disabled  SatFdbkVariant=Disabled  DerivativeFilterVariant=ContFilter  NVariant=InternalParameters  NCopyVariant=Disabled  FilterICVariant=InternalICsFilter  IntegratorICVariant=InternalICs  ExternalResetVariant=Disabled  TRSumVariant=Passthrough  SumFdbkVariant=Disabled  SumVariant=Sum_PID  TsampFilterVariant=InternalTs  TsampNgainVariant=Passthrough  TsampIntegralVariant=Disabled_SignalSpec  ExternalSaturationOutDataTypeStr=Inherit: Same as second input  DerivativeSourceVariant=ErrorSignal  PreIntVariant=InternalPreInt
  PID Controller2 : slpidlib/PID Controller  Controller=PI  Form=Parallel  TimeDomain=Continuous-time  UseExternalTs=off  SampleTime=-1  IntegratorMethod=Forward Euler  FilterMethod=Forward Euler  ControllerParametersSource=internal  P=0.6  I=0.05  UseKiTs=off  D=0  UseExternalDerivativeSource=off  N=100  UseFilter=on  TunerSelectOption=Transfer Function Based (PID Tuner App)  InitialConditionSource=internal  InitialConditionForIntegrator=0  InitialConditionForFilter=0  DifferentiatorICPrevScaledInput=0  ExternalReset=none  TrackingMode=off  Kt=1  LimitOutput=on  SatLimitsSource=internal  UpperSaturationLimit=10*pi/180  LowerSaturationLimit=-10*pi/180  LinearizeAsGain=on  AntiWindupMode=none  Kb=1  LimitIntegrator=off  UpperIntegratorSaturationLimit=inf  LowerIntegratorSaturationLimit=-inf  POutMin=[]  POutMax=[]  IOutMin=[]  IOutMax=[]  DOutMin=[]  DOutMax=[]  NOutMin=[]  NOutMax=[]  SumOutMin=[]  SumOutMax=[]  SaturationOutMin=[]  SaturationOutMax=[]  PParamMin=[]  PParamMax=[]  IParamMin=[]  IParamMax=[]  DParamMin=[]  DParamMax=[]  NParamMin=[]  NParamMax=[]  KbParamMin=[]  KbParamMax=[]  KtParamMin=[]  KtParamMax=[]  KbOutMin=[]  KbOutMax=[]  KtOutMin=[]  KtOutMax=[]  IntegratorOutMin=[]  IntegratorOutMax=[]  FilterOutMin=[]  FilterOutMax=[]  SumI1OutMin=[]  SumI1OutMax=[]  SumI2OutMin=[]  SumI2OutMax=[]  SumI3OutMin=[]  SumI3OutMax=[]  SumI4OutMin=[]  SumI4OutMax=[]  SumDOutMin=[]  SumDOutMax=[]  DifferentiatorOutMin=[]  DifferentiatorOutMax=[]  FilterDiffOutCoefMin=[]  FilterDiffOutCoefMax=[]  ReciprocalOutMin=[]  ReciprocalOutMax=[]  SumDenOutMin=[]  SumDenOutMax=[]  SumNumOutMin=[]  SumNumOutMax=[]  DivideOutMin=[]  DivideOutMax=[]  UdiffTsProdOutMin=[]  UdiffTsProdOutMax=[]  NTsProdOutMin=[]  NTsProdOutMax=[]  UintegralTsProdOutMin=[]  UintegralTsProdOutMax=[]  UngainTsProdOutMin=[]  UngainTsProdOutMax=[]  ClampingZeroOutDataTypeStr=Inherit: Inherit via back propagation  ClampingZeroOutMin=[]  ClampingZeroOutMax=[]  FilterDenConstantOutDataTypeStr=Inherit: Inherit via back propagation  FilterDenConstantOutMin=[]  FilterDenConstantOutMax=[]  PCopyOutDataTypeStr=Inherit: Inherit via back propagation  PCopyOutMin=[]  PCopyOutMax=[]  NCopyOutDataTypeStr=Inherit: Inherit via back propagation  NCopyOutMin=[]  NCopyOutMax=[]  IntegratorContinuousStateAttributes=''  IntegratorStateMustResolveToSignalObject=off  IntegratorRTWStateStorageClass=Auto  FilterContinuousStateAttributes=''  FilterStateMustResolveToSignalObject=off  FilterRTWStateStorageClass=Auto  ParallelPVariant=InternalParameters  IdealPVariant=Disabled  IVariant=InternalParameters  DVariant=Disabled  IntegratorVariant=Continuous  SatVariant=Enabled  AWVariant=Passthrough  PCopyVariant=Disabled  TRVariant=Disabled  FdbkBlocksVariant=Forward  IdealPFdbkVariant=Disabled  SatFdbkVariant=Disabled  DerivativeFilterVariant=Disabled  NVariant=Disabled  NCopyVariant=Disabled_SignalSpec  FilterICVariant=Disabled  IntegratorICVariant=InternalICs  ExternalResetVariant=Disabled  TRSumVariant=Passthrough  SumFdbkVariant=Disabled  SumVariant=Sum_PI  TsampFilterVariant=InternalTs  TsampNgainVariant=Passthrough  TsampIntegralVariant=Disabled_SignalSpec  ExternalSaturationOutDataTypeStr=Inherit: Same as second input  DerivativeSourceVariant=Disabled  PreIntVariant=InternalPreInt
  PID Controller4 : slpidlib/PID Controller  Commented=on  Controller=P  Form=Parallel  TimeDomain=Continuous-time  UseExternalTs=off  SampleTime=-1  IntegratorMethod=Forward Euler  FilterMethod=Forward Euler  ControllerParametersSource=internal  P=-0.00477686409933397  I=1  UseKiTs=off  D=0  UseExternalDerivativeSource=off  N=100  UseFilter=on  TunerSelectOption=Transfer Function Based (PID Tuner App)  InitialConditionSource=internal  InitialConditionForIntegrator=0  InitialConditionForFilter=0  DifferentiatorICPrevScaledInput=0  ExternalReset=none  TrackingMode=off  Kt=1  LimitOutput=on  SatLimitsSource=internal  UpperSaturationLimit=30*(pi/180)  LowerSaturationLimit=-30*(pi/180)  LinearizeAsGain=on  AntiWindupMode=none  Kb=1  LimitIntegrator=off  UpperIntegratorSaturationLimit=inf  LowerIntegratorSaturationLimit=-inf  POutMin=[]  POutMax=[]  IOutMin=[]  IOutMax=[]  DOutMin=[]  DOutMax=[]  NOutMin=[]  NOutMax=[]  SumOutMin=[]  SumOutMax=[]  SaturationOutMin=[]  SaturationOutMax=[]  PParamMin=[]  PParamMax=[]  IParamMin=[]  IParamMax=[]  DParamMin=[]  DParamMax=[]  NParamMin=[]  NParamMax=[]  KbParamMin=[]  KbParamMax=[]  KtParamMin=[]  KtParamMax=[]  KbOutMin=[]  KbOutMax=[]  KtOutMin=[]  KtOutMax=[]  IntegratorOutMin=[]  IntegratorOutMax=[]  FilterOutMin=[]  FilterOutMax=[]  SumI1OutMin=[]  SumI1OutMax=[]  SumI2OutMin=[]  SumI2OutMax=[]  SumI3OutMin=[]  SumI3OutMax=[]  SumI4OutMin=[]  SumI4OutMax=[]  SumDOutMin=[]  SumDOutMax=[]  DifferentiatorOutMin=[]  DifferentiatorOutMax=[]  FilterDiffOutCoefMin=[]  FilterDiffOutCoefMax=[]  ReciprocalOutMin=[]  ReciprocalOutMax=[]  SumDenOutMin=[]  SumDenOutMax=[]  SumNumOutMin=[]  SumNumOutMax=[]  DivideOutMin=[]  DivideOutMax=[]  UdiffTsProdOutMin=[]  UdiffTsProdOutMax=[]  NTsProdOutMin=[]  NTsProdOutMax=[]  UintegralTsProdOutMin=[]  UintegralTsProdOutMax=[]  UngainTsProdOutMin=[]  UngainTsProdOutMax=[]  ClampingZeroOutDataTypeStr=Inherit: Inherit via back propagation  ClampingZeroOutMin=[]  ClampingZeroOutMax=[]  FilterDenConstantOutDataTypeStr=Inherit: Inherit via back propagation  FilterDenConstantOutMin=[]  FilterDenConstantOutMax=[]  PCopyOutDataTypeStr=Inherit: Inherit via back propagation  PCopyOutMin=[]  PCopyOutMax=[]  NCopyOutDataTypeStr=Inherit: Inherit via back propagation  NCopyOutMin=[]  NCopyOutMax=[]  IntegratorContinuousStateAttributes=''  IntegratorStateMustResolveToSignalObject=off  IntegratorRTWStateStorageClass=Auto  FilterContinuousStateAttributes=''  FilterStateMustResolveToSignalObject=off  FilterRTWStateStorageClass=Auto  ParallelPVariant=InternalParameters  IdealPVariant=Disabled  IVariant=Disabled  DVariant=Disabled  IntegratorVariant=Disabled  SatVariant=Enabled  AWVariant=Disabled  PCopyVariant=Disabled  TRVariant=Disabled  FdbkBlocksVariant=Forward  IdealPFdbkVariant=Disabled  SatFdbkVariant=Disabled  DerivativeFilterVariant=Disabled  NVariant=Disabled  NCopyVariant=Disabled_SignalSpec  FilterICVariant=Disabled  IntegratorICVariant=Disabled  ExternalResetVariant=Disabled  TRSumVariant=Passthrough  SumFdbkVariant=Disabled  SumVariant=Passthrough_P  TsampFilterVariant=InternalTs  TsampNgainVariant=Passthrough  TsampIntegralVariant=Disabled_SignalSpec  ExternalSaturationOutDataTypeStr=Inherit: Same as second input  DerivativeSourceVariant=Disabled  PreIntVariant=InternalPreInt
  PID Controller6 : slpidlib/PID Controller  Controller=PI  Form=Parallel  TimeDomain=Continuous-time  UseExternalTs=off  SampleTime=-1  IntegratorMethod=Forward Euler  FilterMethod=Forward Euler  ControllerParametersSource=internal  P=3.44983537526744  I=0.07  UseKiTs=off  D=0  UseExternalDerivativeSource=off  N=100  UseFilter=on  TunerSelectOption=Transfer Function Based (PID Tuner App)  InitialConditionSource=internal  InitialConditionForIntegrator=0  InitialConditionForFilter=0  DifferentiatorICPrevScaledInput=0  ExternalReset=none  TrackingMode=off  Kt=1  LimitOutput=on  SatLimitsSource=internal  UpperSaturationLimit=45*pi/180  LowerSaturationLimit=-45*pi/180  LinearizeAsGain=on  AntiWindupMode=none  Kb=1  LimitIntegrator=off  UpperIntegratorSaturationLimit=inf  LowerIntegratorSaturationLimit=-inf  POutMin=[]  POutMax=[]  IOutMin=[]  IOutMax=[]  DOutMin=[]  DOutMax=[]  NOutMin=[]  NOutMax=[]  SumOutMin=[]  SumOutMax=[]  SaturationOutMin=[]  SaturationOutMax=[]  PParamMin=[]  PParamMax=[]  IParamMin=[]  IParamMax=[]  DParamMin=[]  DParamMax=[]  NParamMin=[]  NParamMax=[]  KbParamMin=[]  KbParamMax=[]  KtParamMin=[]  KtParamMax=[]  KbOutMin=[]  KbOutMax=[]  KtOutMin=[]  KtOutMax=[]  IntegratorOutMin=[]  IntegratorOutMax=[]  FilterOutMin=[]  FilterOutMax=[]  SumI1OutMin=[]  SumI1OutMax=[]  SumI2OutMin=[]  SumI2OutMax=[]  SumI3OutMin=[]  SumI3OutMax=[]  SumI4OutMin=[]  SumI4OutMax=[]  SumDOutMin=[]  SumDOutMax=[]  DifferentiatorOutMin=[]  DifferentiatorOutMax=[]  FilterDiffOutCoefMin=[]  FilterDiffOutCoefMax=[]  ReciprocalOutMin=[]  ReciprocalOutMax=[]  SumDenOutMin=[]  SumDenOutMax=[]  SumNumOutMin=[]  SumNumOutMax=[]  DivideOutMin=[]  DivideOutMax=[]  UdiffTsProdOutMin=[]  UdiffTsProdOutMax=[]  NTsProdOutMin=[]  NTsProdOutMax=[]  UintegralTsProdOutMin=[]  UintegralTsProdOutMax=[]  UngainTsProdOutMin=[]  UngainTsProdOutMax=[]  ClampingZeroOutDataTypeStr=Inherit: Inherit via back propagation  ClampingZeroOutMin=[]  ClampingZeroOutMax=[]  FilterDenConstantOutDataTypeStr=Inherit: Inherit via back propagation  FilterDenConstantOutMin=[]  FilterDenConstantOutMax=[]  PCopyOutDataTypeStr=Inherit: Inherit via back propagation  PCopyOutMin=[]  PCopyOutMax=[]  NCopyOutDataTypeStr=Inherit: Inherit via back propagation  NCopyOutMin=[]  NCopyOutMax=[]  IntegratorContinuousStateAttributes=''  IntegratorStateMustResolveToSignalObject=off  IntegratorRTWStateStorageClass=Auto  FilterContinuousStateAttributes=''  FilterStateMustResolveToSignalObject=off  FilterRTWStateStorageClass=Auto  ParallelPVariant=InternalParameters  IdealPVariant=Disabled  IVariant=InternalParameters  DVariant=Disabled  IntegratorVariant=Continuous  SatVariant=Enabled  AWVariant=Passthrough  PCopyVariant=Disabled  TRVariant=Disabled  FdbkBlocksVariant=Forward  IdealPFdbkVariant=Disabled  SatFdbkVariant=Disabled  DerivativeFilterVariant=Disabled  NVariant=Disabled  NCopyVariant=Disabled_SignalSpec  FilterICVariant=Disabled  IntegratorICVariant=InternalICs  ExternalResetVariant=Disabled  TRSumVariant=Passthrough  SumFdbkVariant=Disabled  SumVariant=Sum_PI  TsampFilterVariant=InternalTs  TsampNgainVariant=Passthrough  TsampIntegralVariant=Disabled_SignalSpec  ExternalSaturationOutDataTypeStr=Inherit: Same as second input  DerivativeSourceVariant=Disabled  PreIntVariant=InternalPreInt
  Saturation : Saturate  UpperLimit=5*pi/180  LowerLimit=-5*pi/180
  Sum : Sum  Commented=on  Inputs=|+-
  Sum1 : Sum  Commented=on  Inputs=|+-
  Sum2 : Sum  Inputs=|+-
  Sum4 : Sum  Commented=on  Inputs=|+-
  Sum5 : Sum  Inputs=|+-
  airspeed : Outport
  ele : Outport  Port=2
  rud : Outport  Port=3
  ail : Outport  Port=4
  wires:
  Sum1/1 -> PID Controller1/1
  Sum5/1 -> PID Controller6/1
  theta/1 -> Sum1/2
  H2D/1 -> Sum4/1
  U/1 -> Sum4/2
  Sum/1 -> PID Controller/1
  PID Controller1/1 -> Sum/1
  Sum4/1 -> PID Controller4/1
  PID Controller4/1 -> Sum1/1
  phi/1 -> Sum5/2
  q/1 -> Sum/2
  speed/1 -> airspeed/1
  Saturation/1 -> rud/1
  Gain/1 -> Saturation/1
  Sum2/1 -> PID Controller2/1
  p/1 -> Sum2/2
  PID Controller6/1 -> Sum2/1
  Gain1/1 -> Sum5/1
  PID Controller2/1 -> ail/1, Gain/1
  action/1 -> Gain2/1
  Gain2/1 -> Gain1/1
  Gain3/1 -> Gain4/1
  Gain4/1 -> H2D/1
  Constant/1 -> ele/1

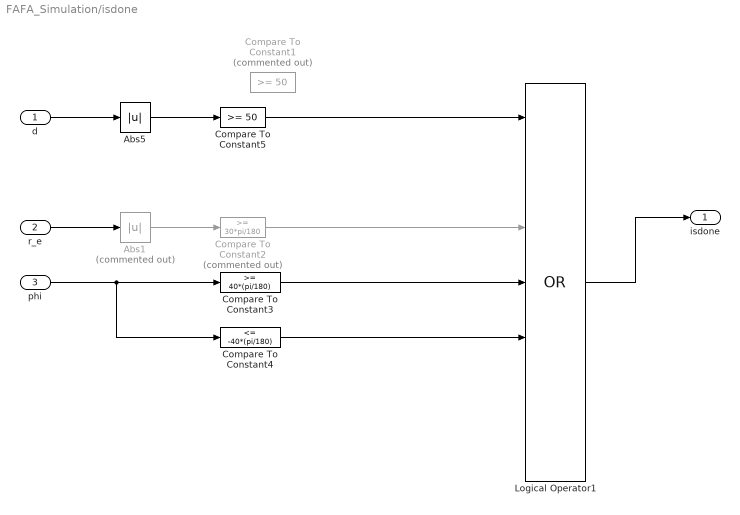
== system FAFA_Simulation/isdone ==
  d : Inport
  r_e : Inport  Port=2
  phi : Inport  Port=3
  Abs1 : Abs  Commented=on  SaturateOnIntegerOverflow=off
  Abs5 : Abs  SaturateOnIntegerOverflow=off
  Compare To Constant1 : simulink/Logic and Bit Operations/Compare To Constant  Commented=on  relop=>=  const=50  OutDataTypeStr=boolean
  Compare To Constant2 : simulink/Logic and Bit Operations/Compare To Constant  Commented=on  relop=>=  const=30*pi/180  OutDataTypeStr=boolean
  Compare To Constant3 : simulink/Logic and Bit Operations/Compare To Constant  relop=>=  const=40*(pi/180)  OutDataTypeStr=boolean
  Compare To Constant4 : simulink/Logic and Bit Operations/Compare To Constant  relop=<=  const=-40*(pi/180)  OutDataTypeStr=boolean
  Compare To Constant5 : simulink/Logic and Bit Operations/Compare To Constant  relop=>=  const=50  OutDataTypeStr=boolean
  Logical Operator1 : Logic  Operator=OR  Inputs=7  AllPortsSameDT=off  OutDataTypeStr=boolean
  isdone : Outport
  wires:
  d/1 -> Abs5/1
  Abs5/1 -> Compare To Constant5/1
  Logical Operator1/1 -> isdone/1
  Compare To Constant5/1 -> Logical Operator1/1
  phi/1 -> Compare To Constant4/1, Compare To Constant3/1
  Compare To Constant3/1 -> Logical Operator1/4
  Compare To Constant4/1 -> Logical Operator1/5
  r_e/1 -> Abs1/1
  Abs1/1 -> Compare To Constant2/1
  Compare To Constant2/1 -> Logical Operator1/3

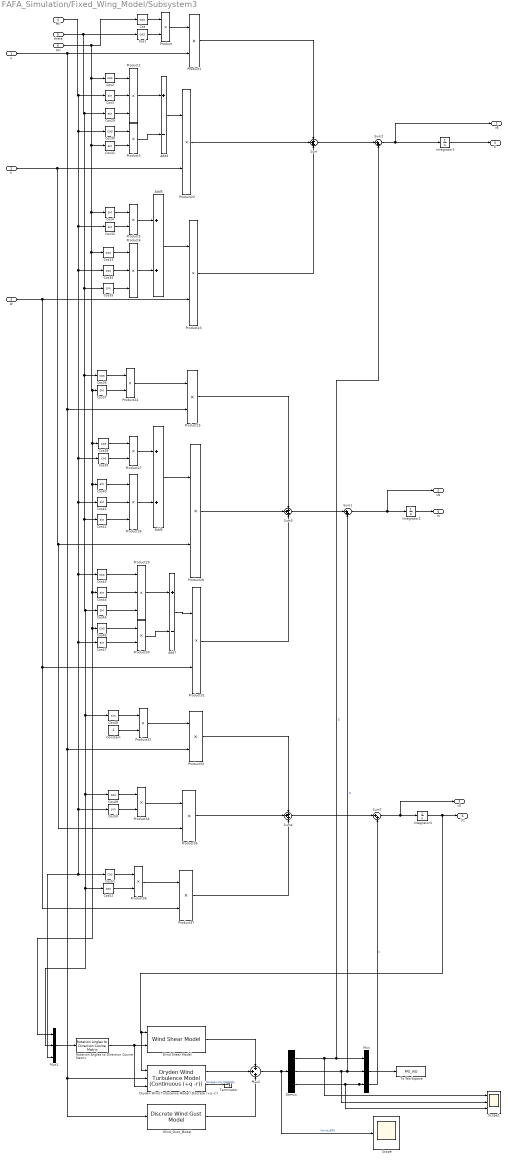
== system FAFA_Simulation/Fixed_Wing_Model/Subsystem3 ==
  u : Inport
  V : Inport  Port=2
  W : Inport  Port=3
  Phi : Inport  Port=4
  theta : Inport  Port=5
  psi : Inport  Port=6
  Add4 : Sum  Inputs=+-
  Add5 : Sum
  Add6 : Sum
  Add7 : Sum  Inputs=+-
  Constant : Constant  Value=-1
  Cos{,1..2,30,33..34,36,38..39,43,46,49,51..52} (14 alike) : Trigonometry  Operator=cos
  Cos{3..4,29,31..32,35,37,40..42,44..45,47..48,50} (15 alike) : Trigonometry
  Demux : Demux  Outputs=3
  Dryden Wind Turbulence Model (Discrete (+q -r)) : aerolibwind2/Dryden Wind Turbulence Model  (Continuous (+q -r))  units=Metric (MKS)  spec=MIL-F-8785C  model=Continuous Dryden (+q -r)  W20=wind_turbulance_value0  Wdeg=1  TurbProb=10^-2 - Light  L_high=533.4  Wingspan=2  ts=0.1  Seed=[23341 23342 23343 23344]  T_on=on
  Integrator1 : Integrator  InitialCondition=E
  Integrator2 : Integrator  InitialCondition=N
  Integrator3 : Integrator  InitialCondition=U
  Mux : Mux  Inputs=3
  Mux1 : Mux  Inputs=[1 1 1]
  Plus2 : Sum  Inputs=+++
  Product{,1,3,5,22..25,27..28,30..37} (18 alike) : Product
  Product{2,4,26,29} (4 alike) : Product  Inputs=3
  Rotation Angles to Direction Cosine Matrix : sharedtransform/Rotation Angles to Direction Cosine Matrix  rotationOrder=ZYX  aMode=aMode
  Scope : Scope
  Scope1 : Scope  NumInputPorts=3
  Sum : Sum  Inputs=+++
  Sum1 : Sum  Inputs=|++
  Sum2 : Sum  Inputs=|++
  Sum3 : Sum  Inputs=+++
  Sum4 : Sum  Inputs=+++
  Sum7 : Sum  Inputs=|++
  Terminator : Terminator
  To Workspace : ToWorkspace  VariableName=PPO_WD  SaveFormat=Timeseries  SampleTime=-1
  Wind Shear Model : aerolibwind2/Wind Shear Model  units=Metric (MKS)  phase=Category C - Terminal Flight Phase  W_20=wind_value0  Wdeg=90.90401785714285
  Wind_Gust_Model : aerolibwind2/Discrete Wind Gust Model  units=Metric (MKS)  Gx=on  Gy=on  Gz=off  t_0=5  d_m=[120 120 80]  v_m=[wind_E0,wind_N0,10]
  vE : Outport
  vN : Outport  Port=2
  vU : Outport  Port=3
  E : Outport  Port=4
  N : Outport  Port=5
  U1 : Outport  Port=6
  wires:
  Cos/1 -> Product/1
  Cos1/1 -> Product/2
  Product/1 -> Product1/1
  Cos2/1 -> Product2/1
  Cos3/1 -> Product2/2
  Product1/1 -> Sum/1
  Product22/1 -> Sum/2
  Integrator1/1 -> E/1
  Integrator2/1 -> N/1
  psi/1 -> Mux1/1, Cos46/1, Cos44/1, Cos40/1, Cos38/1, Cos37/1, Cos33/1, Cos4/1, Cos31/1, Cos2/1, Cos/1
  theta/1 -> Cos48/1, Mux1/2, Cos52/1, Cos49/1, Cos45/1, Cos42/1, Cos36/1, Cos35/1, Cos29/1, Cos1/1
  u/1 -> Wind_Gust_Model/1, Dryden Wind Turbulence Model (Discrete (+q -r))/2, Product33/2, Product25/2, Product1/2
  Cos29/1 -> Product2/3
  Product2/1 -> Add4/1
  Phi/1 -> Cos51/1, Mux1/3, Cos50/1, Cos47/1, Cos43/1, Cos41/1, Cos39/1, Cos34/1, Cos32/1, Cos30/1, Cos3/1
  Product3/1 -> Add4/2
  Cos31/1 -> Product3/2
  Cos30/1 -> Product3/1
  Add4/1 -> Product22/1
  V/1 -> Product35/2, Product28/2, Product22/2
  W/1 -> Product37/2, Product31/2, Product23/2
  Cos4/1 -> Product5/1
  Cos32/1 -> Product5/2
  Cos33/1 -> Product4/1
  Cos34/1 -> Product4/2
  Cos35/1 -> Product4/3
  Product4/1 -> Add5/2
  Product5/1 -> Add5/1
  Add5/1 -> Product23/1
  Product23/1 -> Sum/3
  Product24/1 -> Product25/1
  Cos36/1 -> Product24/1
  Cos37/1 -> Product24/2
  Product27/1 -> Add6/1
  Product26/1 -> Add6/2
  Cos38/1 -> Product27/1
  Cos39/1 -> Product27/2
  Cos41/1 -> Product26/2
  Cos42/1 -> Product26/3
  Cos40/1 -> Product26/1
  Add6/1 -> Product28/1
  Product30/1 -> Add7/2
  Product29/1 -> Add7/1
  Cos43/1 -> Product29/1
  Cos44/1 -> Product29/2
  Cos45/1 -> Product29/3
  Cos46/1 -> Product30/1
  Cos47/1 -> Product30/2
  Add7/1 -> Product31/1
  Product28/1 -> Sum3/2
  Product25/1 -> Sum3/1
  Product31/1 -> Sum3/3
  Cos48/1 -> Product32/1
  Constant/1 -> Product32/2
  Product32/1 -> Product33/1
  Cos49/1 -> Product34/1
  Cos50/1 -> Product34/2
  Product34/1 -> Product35/1
  Cos51/1 -> Product36/1
  Product36/1 -> Product37/1
  Cos52/1 -> Product36/2
  Product35/1 -> Sum4/2
  Product33/1 -> Sum4/1
  Product37/1 -> Sum4/3
  Integrator3/1 -> Dryden Wind Turbulence Model (Discrete (+q -r))/1, Wind Shear Model/1, U1/1
  Mux1/1 -> Rotation Angles to Direction Cosine Matrix/1
  Rotation Angles to Direction Cosine Matrix/1 -> Dryden Wind Turbulence Model (Discrete (+q -r))/3, Wind Shear Model/2
  Sum7/1 -> vU/1, Integrator3/1
  Sum4/1 -> Sum7/1
  Sum3/1 -> Sum1/1
  Sum1/1 -> vN/1, Integrator2/1
  Sum/1 -> Sum2/1
  Sum2/1 -> vE/1, Integrator1/1
  Dryden Wind Turbulence Model (Discrete (+q -r))/1 -> Plus2/2
  Wind Shear Model/1 -> Plus2/1
  Wind_Gust_Model/1 -> Plus2/3
  Dryden Wind Turbulence Model (Discrete (+q -r))/2 -> Terminator/1  "Omegawind_UAVbody"
  Plus2/1 -> Scope/1, Demux/1  "Vwind_ENU"
  Demux/2 -> Scope1/2, Mux/2, Sum1/2  "N"
  Demux/3 -> Scope1/3, Sum7/2, Mux/3  "U"
  Mux/1 -> To Workspace/1
  Demux/1 -> Scope1/1, Sum2/2, Mux/1  "E"

== matlab function FAFA_Simulation/OBSERVATION/MATLAB Function6 ==
  data: x input; y output; finite input
function y = Normalization(x,finite)
y = (x-(-finite))/(finite-(-finite))*2-1;

== matlab function FAFA_Simulation/OBSERVATION/MATLAB Function7 ==
  data: x input; y output; finite input
function y = Normalization(x,finite)
y = (x-(-finite))/(finite-(-finite))*2-1;
